simulink model "RoadsterHover"  (R2025b)
settings: Solver=ode1  StartTime=0.0  StopTime=8  FixedStep=1e-3  RelTol=1e-3
undefined symbols (not defined in the file): rtl
Description:
  | Hover on the 4 lift thrusters. Logged: y, vy, F_lift, P_tank, T_tank, m_air, phase, Isp. Phases: 0 climb, 1 hold, 2 descend, 3 landed.
settings Model: Creator=kichuiyer  LastModifiedBy=kichuiyer
settings DataIOCC: SaveOutput=off

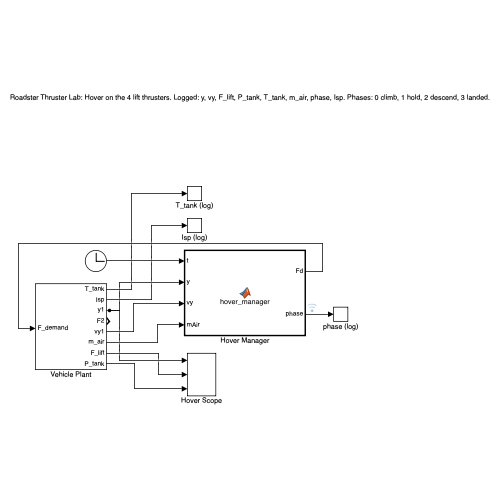
[thumbnail: Simulink's stored preview of the top-level diagram]
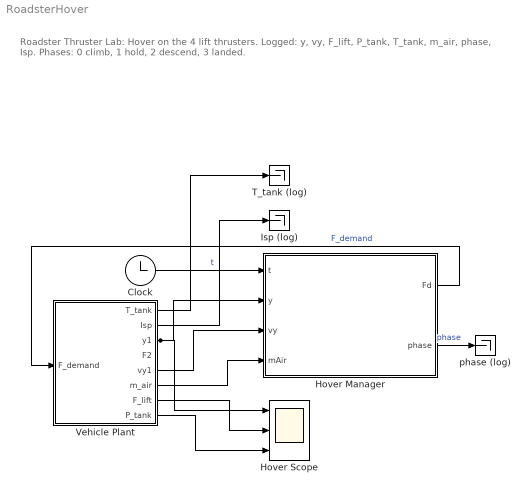
== system RoadsterHover ==
  note: Roadster Thruster Lab: Hover on the 4 lift thrusters. Logged: y, vy, F_lift, P_tank, T_tank, m_air, phase, Isp. Phases: 0 climb, 1 hold, 2 descend, 3 landed.
  Clock : Clock
  Hover Manager : MATLAB Function  TreatAsAtomicUnit=on
  Hover Scope : Scope  NumInputPorts=3
  Isp (log) : Terminator
  T_tank (log) : Terminator
  Vehicle Plant : Subsystem
  phase (log) : Terminator
  wires:
  Vehicle Plant/6(m_air) -> Hover Manager/4(mAir)
  Vehicle Plant/3(y1) -> Hover Manager/2(y), Hover Scope/1
  Vehicle Plant/8(P_tank) -> Hover Scope/3
  Vehicle Plant/1(T_tank) -> T_tank (log)/1
  Hover Manager/2(phase) -> phase (log)/1  "phase"
  Vehicle Plant/5(vy1) -> Hover Manager/3(vy)
  Vehicle Plant/2(Isp) -> Isp (log)/1
  Hover Manager/1(Fd) -> Vehicle Plant/1(F_demand)  "F_demand"
  Vehicle Plant/7(F_lift) -> Hover Scope/2
  Clock/1 -> Hover Manager/1(t)  "t"

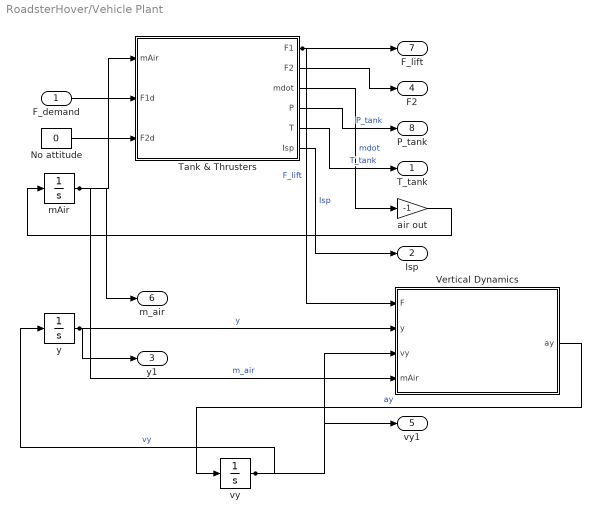
== system RoadsterHover/Vehicle Plant ==
  F_demand : Inport
  No attitude : Constant  Value=0
  Tank & Thrusters : MATLAB Function  TreatAsAtomicUnit=on
  Vertical Dynamics : MATLAB Function  TreatAsAtomicUnit=on
  air out : Gain  Gain=-1
  mAir : Integrator  InitialCondition=rtl.m0  LimitOutput=on  LowerSaturationLimit=0
  vy : Integrator
  y : Integrator  LimitOutput=on  LowerSaturationLimit=0
  T_tank : Outport
  Isp : Outport  Port=2
  y1 : Outport  Port=3
  F2 : Outport  Port=4
  vy1 : Outport  Port=5
  m_air : Outport  Port=6
  F_lift : Outport  Port=7
  P_tank : Outport  Port=8
  wires:
  Tank & Thrusters/6(Isp) -> Isp/1  "Isp"
  Tank & Thrusters/4(P) -> P_tank/1  "P_tank"
  Tank & Thrusters/3(mdot) -> air out/1  "mdot"
  air out/1 -> mAir/1
  y/1 -> y1/1, Vertical Dynamics/2(y)  "y"
  vy/1 -> Vertical Dynamics/3(vy), vy1/1, y/1  "vy"
  Vertical Dynamics/1(ay) -> vy/1  "ay"
  mAir/1 -> Tank & Thrusters/1(mAir), m_air/1, Vertical Dynamics/4(mAir)  "m_air"
  Tank & Thrusters/5(T) -> T_tank/1  "T_tank"
  Tank & Thrusters/2(F2) -> F2/1
  Tank & Thrusters/1(F1) -> F_lift/1, Vertical Dynamics/1(F)  "F_lift"
  No attitude/1 -> Tank & Thrusters/3(F2d)
  F_demand/1 -> Tank & Thrusters/2(F1d)

== matlab function RoadsterHover/Vehicle Plant/Tank & Thrusters ==
  data: mAir input; F1 output; F1d input; F2d input; F2 output; mdot output; P output; T output; Isp output; rtl parameter
function [F1, F2, mdot, P, T, Isp] = tank_thrusters(mAir, F1d, F2d, rtl)
%#codegen
% Cold-gas tank with adiabatic blowdown feeding regulated, choked nozzles.
r   = max(mAir, 1e-6) / rtl.m0;
P   = rtl.P0 * r^rtl.gam;              % isentropic: gas left behind expands
T   = rtl.T0 * r^(rtl.gam - 1);        % ...and cools
pc  = min(rtl.Preg, P);                % regulator caps the nozzle feed
Cf  = rtl.CFm + (pc*rtl.PR - rtl.Pa)/pc*rtl.eps;
Isp = Cf * sqrt(rtl.R*T/rtl.gam) / rtl.CK / rtl.g0;
k   = pc / rtl.Preg;
if pc < 15e5, k = 0; end               % too little pressure to run
F1  = max(F1d, 0) * k;
F2  = max(F2d, 0) * k;
mdot = (F1 + F2) / (Isp * rtl.g0);     % rocket equation: mdot = F/(Isp g0)

== matlab function RoadsterHover/Hover Manager ==
  settings: updateMethod=DISCRETE  sampleTime=1e-3
  data: t input; Fd output; y input; vy input; mAir input; phase output; rtl parameter
function [Fd, phase] = hover_manager(t, y, vy, mAir, rtl)
%#codegen
% Climb to the target height, hold, then descend under control once the tank
% nears the regulator pressure so there is still air left to land.
persistent ph tgt
if isempty(ph), ph = 0; tgt = rtl.hoverAlt; end   % 0 climb, 1 hold, 2 descend, 3 landed
P = rtl.P0*(max(mAir, 1e-6)/rtl.m0)^rtl.gam;
if (ph == 0 || ph == 1) && P < 1.08*rtl.Preg, ph = 2; end
if ph == 0 && y >= 0.95*rtl.hoverAlt, ph = 1; end
vref = 0;
if ph == 2
    tgt = max(0, tgt - 0.9*1e-3);
    if tgt > 0, vref = -0.9; end
    if y <= 0 && t > 0.5, ph = 3; end
end
Fd = 0;
if ph < 3
    m = rtl.dry + mAir;
    Fd = min(rtl.FliftMax, max(0, m*(rtl.g0 + 4*(tgt - y) + 4.5*(vref - vy))));
end
phase = ph;

== matlab function RoadsterHover/Vehicle Plant/Vertical Dynamics ==
  data: F input; ay output; y input; vy input; mAir input; rtl parameter
function ay = vertical_dynamics(F, y, vy, mAir, rtl)
%#codegen
ay = F/(rtl.dry + mAir) - rtl.g0;
if y <= 1e-9 && ay < 0
    ay = 0;
    if vy < 0, ay = -vy/1e-3; end   % ground stops the car
end
